simulink model "reachout_sample"  (Simulink 8.1)
settings: Solver=ode4  SolverMode=SingleTasking  StartTime=0.0  StopTime=inf  FixedStep=0.0005  RelTol=1e-3
model workspace (MAT data in the model file):
  BKIN_STEP_TIME = 0.0005
  col_x = 1
  col_y = 2
  E_STAY_CENTER = 2
  E_TARGET_ON = 3
  E_HOLD_AT_TARGET = 5
  VRAD = 3
  LRAD = 4
  INIT_COLOR = 5
  REACH_COLOR = 6
  SHOULDER_VISC = 1
  ELBOW_VISC = 2
  START_TARGET = 1
  LOAD = 3
  DELAY_1ST_TARGET_FIXED = 4
  DELAY_1ST_TARGET_RANDOM = 5
  MAX_REACH_TIME = 6
  DELAY_2ND_TARGET = 7
  DELAY_POST_TRIAL = 8
  END_TARGET = 2
  A_VISC = 3
  B_VISC = 4
  C_VISC = 5
  D_VISC : num (value not decoded)
StartFcn:
  |  warndlg('Dexterit-E models cannot run under simulation. Please compile your model and run it from within Dexterit-E.');set_param(bdroot,'SimulationCommand','stop')
libraries: General x3, KINARM_loads x3, Video x3, KINARM_general x2, KINARM_EP_loads x2
CloseFcn:
  | rtwprivate ssgencode ModelCloseRequest b2lab2d
settings Model: Creator=Chris Grebeldinger  LastModifiedBy=BKIN TECHNOLOGIES  ModifiedComment=chris -- Wed Feb 16 09:18:30 2005 -- Version 1.1384  ModifiedHistory=Feb 16/05 - Add error repeat, add offset ramp  ExtModeArmWhenConnect=off  ExtModeLogAll=off  BufferReuse=off
settings DataIOCC: LimitDataPoints=off  SaveOutput=off  SaveTime=off  SignalLoggingName=sigsOut
settings OptimizationCC: BlockReduction=off  BooleanDataType=off  OptimizeBlockIOStorage=off  BufferReuse=off  ExpressionFolding=off  FoldNonRolledExpr=off  LocalBlockOutputs=off  InitFltsAndDblsToZero=on
settings DebuggingCC: SaveWithParameterizedLinksMsg=none  SignalResolutionControl=TryResolveAllWithWarning  SolverPrmCheckMsg=none  MultiTaskDSMMsg=warning  MultiTaskCondExecSysMsg=none  StrictBusMsg=Warning
settings HardwareCC: ProdIntDivRoundTo=Zero  ProdEndianess=LittleEndian  ProdHWDeviceType=Generic->32-bit x86 compatible  TargetHWDeviceType=32-bit Generic
settings SFSimCC: SimCustomHeaderCode="#include \"stdlib.h\""  SFSimEcho=off  SimParseCustomCode=off
settings RTWCC: SystemTargetFile=xpctarget.tlc  TemplateMakefile=xpc_default_tmf  Description=xPC Target  ProcessScript=xpctarget_make_rtw_hook  CustomSourceCode="#include \"stdlib.h\""  IncludeERTFirstTime=on  RTWCompilerOptimization=On
settings CodeAppCC: MaxIdLength=63
settings xpcTargetCC: TargetFcnLib=ansi_tfl_tmw.mat  CodeReplacementLibrary=XPC_BLAS  ParMdlRefBuildCompliant=on  ConcurrentExecutionCompliant=on  CombineSignalStateStructs=off  MATLABClassNameForMDSCustomization=xpcAperiodicCustomization  GRTInterface=on  GenerateAllocFcn=off  xPCTaskExecutionProfile=off  xPCRL32EventNumber=5000  xPCisDownloadable=off  xPCisDefaultEnv=off  xPCLoadParamSetFile=off  xPCConcurrentTasks=off  xPCEnableSFAnimation=off

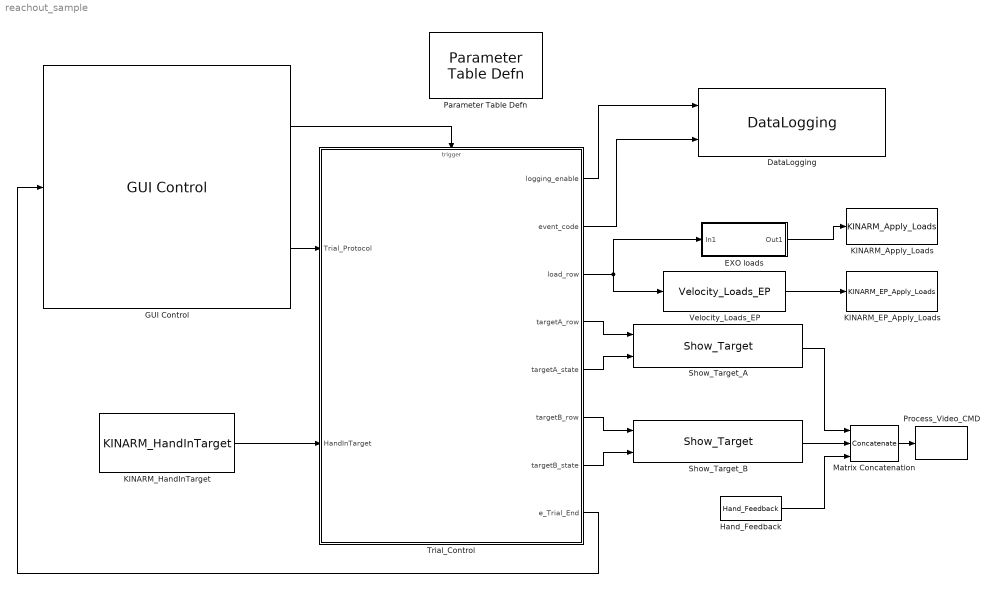
== system reachout_sample ==
  DataLogging : General/DataLogging  log_event_codes=on  log_analog_inputs=off
      link override Poll KINARM/EPTorqueCMD: GotoTag=KINARMEPTorqueCMD
      link override Poll KINARM/TorqueCMD: GotoTag=KINARMTorqueCMD
  EXO loads : Subsystem
  GUI Control : General/GUI Control  target_type_str=Circle  Target_Type=1  XYcols=[1 2]  Vcols=3  Lcols=4  indices_padding=[0 0 0 0;0 0 0 0]  task_version=1.0  show_repeat_trial_flag=off
  Hand_Feedback : KINARM_general/Hand_Feedback  feedback_cntl_src=none
  KINARM_Apply_Loads : KINARM_loads/KINARM_Apply_Loads  up_duration=0  down_duration=0  max_torque=13
  KINARM_EP_Apply_Loads : KINARM_EP_loads/KINARM_EP_Apply_Loads  up_duration=1500  down_duration=1500  max_force=60
  KINARM_HandInTarget : KINARM_general/KINARM_HandInTarget  use_dominant_hand=on  target_type=Circle  num_states=1  attribcol1=[4]  attribcol2=[4]  attribcol3=[5]  attribcol4=[6]  attribcol5=[0]
  Matrix Concatenation : Concatenate  NumInputs=3  Mode=Multidimensional array
  Parameter Table Defn : General/Parameter Table Defn  ShowInLibBrowser=0
  Process_Video_CMD : Video/Process_Video_CMD
  Show_Target_A : Video/Show_Target  target_type=Circle  num_states=2  attribcol1=[INIT_COLOR 0 0 VRAD]  attribcol2=[REACH_COLOR 0 0 VRAD]  attribcol3=[0 0 0 0]  attribcol4=[0 0 0 0]  attribcol5=[0 0 24 0]  stateindices_padding=[0 0 0 0 0 0 0;0 0 0 0 0 0 0;0 0 0 0 0 0 0;0 0 0 0 0 0 0;0 0 0 0 0 0 0]  source=dialog  opacity=100  target_display=Both subject and operator displays  num_col=4
  Show_Target_B : Video/Show_Target  target_type=Circle  num_states=2  attribcol1=[INIT_COLOR 0 0 VRAD]  attribcol2=[REACH_COLOR 0 0 VRAD]  attribcol3=[0 0 0 0]  attribcol4=[0 0 0 0]  attribcol5=[0 0 24 0]  stateindices_padding=[0 0 0 0 0 0 0;0 0 0 0 0 0 0;0 0 0 0 0 0 0;0 0 0 0 0 0 0;0 0 0 0 0 0 0]  source=dialog  opacity=100  target_display=Both subject and operator displays  num_col=4
  Trial_Control : Stateflow chart  TreatAsAtomicUnit=on
  Velocity_Loads_EP : KINARM_EP_loads/Velocity_Loads_EP  use_dom_hand=on  loadcol=[A_VISC B_VISC C_VISC D_VISC]  source=dialog  scaling=1  stability=on
  wires:
  KINARM_HandInTarget/1 -> Trial_Control/2(HandInTarget)
  Show_Target_A/1 -> Matrix Concatenation/1
  GUI Control/2 -> Trial_Control/1(Trial_Protocol)
  Trial_Control/8(e_Trial_End) -> GUI Control/1
  GUI Control/1 -> Trial_Control/Trigger
  Trial_Control/5(targetA_state) -> Show_Target_A/2
  Trial_Control/4(targetA_row) -> Show_Target_A/1
  Matrix Concatenation/1 -> Process_Video_CMD/1
  Hand_Feedback/1 -> Matrix Concatenation/3
  Show_Target_B/1 -> Matrix Concatenation/2
  Trial_Control/6(targetB_row) -> Show_Target_B/1
  Trial_Control/7(targetB_state) -> Show_Target_B/2
  Trial_Control/3(load_row) -> Velocity_Loads_EP/1, EXO loads/1(In1)
  Trial_Control/1(logging_enable) -> DataLogging/1
  Trial_Control/2(event_code) -> DataLogging/2
  EXO loads/1(Out1) -> KINARM_Apply_Loads/1
  Velocity_Loads_EP/1 -> KINARM_EP_Apply_Loads/1

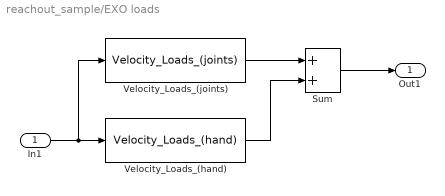
== system reachout_sample/EXO loads ==
  In1 : Inport
  Sum : Sum
  Velocity_Loads_(hand) : KINARM_loads/Velocity_Loads_(hand)  use_dom_hand=on  loadcol=[A_VISC B_VISC C_VISC D_VISC]  source=dialog  scaling=1  stability=on
  Velocity_Loads_(joints) : KINARM_loads/Velocity_Loads_(joints)  use_dom_hand=on  loadcol=[SHOULDER_VISC 0 0 ELBOW_VISC]  source=dialog  scaling=1  stability=on
  Out1 : Outport
  wires:
  In1/1 -> Velocity_Loads_(joints)/1, Velocity_Loads_(hand)/1
  Sum/1 -> Out1/1
  Velocity_Loads_(joints)/1 -> Sum/1
  Velocity_Loads_(hand)/1 -> Sum/2

== stateflow chart Trial_Control ==
  settings: sampleTime=0.001
  state Inter_Trial_State/
    // Turn off both targets, turn off data logging, reset the
    // event code, and send the e_Trial_End Stateflow event.
    event_code = 0;
    targetA_state = 0;
    targetB_state = 0;
    logging_enable = 0;
    e_Trial_End;
  state Initialize/
    // Both the targets and data logging are initially off.
    targetA_state = 0;
    targetB_state = 0;
    logging_enable = 0;
  state MainTrial
    state ShowSecondTarget/
      // Turn on second target and log an event indicating this has occurred. Then wait until the hand is the target or until a specified time has elapsed.
      event_code = E_TARGET_ON;
      targetB_row = Trial_Protocol[END_TARGET];
      targetB_state = 1;
      tickCount = Trial_Protocol[MAX_REACH_TIME];
    state StayAtSecondTarget/
      // Log an event that the second target was reached, change that target's state, and then wait for a specified time.
      event_code = E_HOLD_AT_TARGET;
      targetB_state = 2;
      tickCount = Trial_Protocol[DELAY_2ND_TARGET];
    state EndOfTrial/
      // Set the post-trial delay.
      tickCount = Trial_Protocol[DELAY_POST_TRIAL];
    state StayAtFirstTarget/
      // Log an event that target was reached, begin data logging, change the first target's state, and then wait for a specified time.
      // The wait time may have both a fixed and a random component. The hand must stay in the target for the full wait time.
      logging_enable = 1;
      event_code = E_STAY_CENTER;
      targetA_state = 2;
      tickCount = Trial_Protocol[DELAY_1ST_TARGET_FIXED] + Trial_Protocol[DELAY_1ST_TARGET_RANDOM] * rand() / RAND_MAX;
    state ShowFirstTarget/
      // Turn on first target, set loading conditions, enable data logging, and wait for a specified time or until the hand is in the target.
      targetA_row = Trial_Protocol[START_TARGET];
      targetA_state = 1;
      load_row = Trial_Protocol[LOAD];
    ShowFirstTarget -> StayAtFirstTarget : [HandInTarget[targetA_row] == 1]
    StayAtFirstTarget -> ShowFirstTarget [order 2] : [HandInTarget[targetA_row] == 0]
    StayAtFirstTarget -> ShowSecondTarget [order 1] : after(tickCount, e_clk)
    ShowSecondTarget -> StayAtSecondTarget [order 2] : [HandInTarget[targetB_row]==1]
    ShowSecondTarget -> EndOfTrial [order 1] : after(tickCount, e_clk)
    StayAtSecondTarget -> EndOfTrial : after(tickCount, e_clk)
  (default) -> Initialize
  Initialize -> ShowFirstTarget
  Inter_Trial_State -> ShowFirstTarget : after(tickCount, e_clk)
  MainTrial -> Inter_Trial_State : e_ExitTrialNow/
      | tickCount = 1;
  EndOfTrial -> Inter_Trial_State
  data: logging_enable output boolean; Trial_Protocol input double; HandInTarget input double; event_code output uint16 [0..] =0; load_row output double [1..32]; targetA_row output double [1..32]; targetA_state output double; targetB_row output double; targetB_state output double; tickCount local double; RAND_MAX constant double =32767
  data load_row settings: description=current index into the loadtable
  data targetA_row settings: description=index of the row currently being used in the TargetTable
  events: e_clk input RISING_EDGE_EVENT; e_ExitTrialNow input EITHER_EDGE_EVENT; e_Trial_End output EITHER_EDGE_EVENT
